simulink model "L3_POLI_ZEROURI_DISCRET"  (R2025b)
settings: Solver=FixedStepDiscrete  StartTime=0.0  StopTime=20  FixedStep=0.1  RelTol=1e-3
settings Model: Creator=elisa  LastModifiedBy=elisa

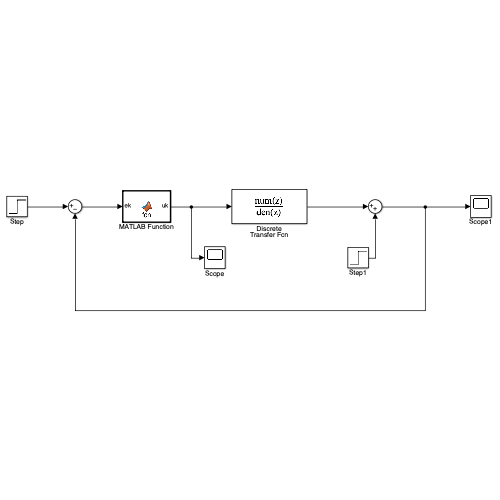
[thumbnail: Simulink's stored preview of the top-level diagram]
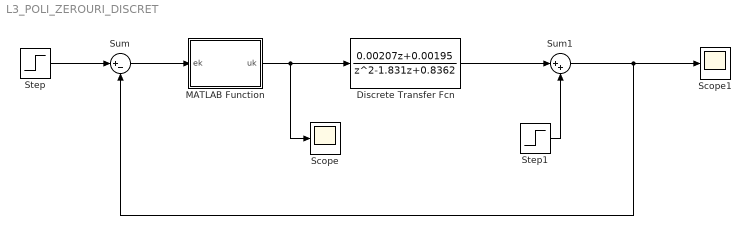
== system L3_POLI_ZEROURI_DISCRET ==
  Discrete Transfer Fcn : DiscreteTransferFcn  Numerator=[0.00207 0.00195]  Denominator=[1 -1.831 0.8362]
  MATLAB Function : MATLAB Function  TreatAsAtomicUnit=on
  Scope : Scope
      settings: ActiveDisplayYMinimum=124.44458746450584  ActiveDisplayYMaximum=170.78058144450188
  Scope1 : Scope
      settings: ActiveDisplayYMinimum=-2.7858479065643103  ActiveDisplayYMaximum=125.07263115907882
  Step : Step  Time=0  After=110  SampleTime=0.1
  Step1 : Step  Time=0  After=10  SampleTime=0.1
  Sum : Sum  Inputs=|+-
  Sum1 : Sum  Inputs=|++
  wires:
  Step/1 -> Sum/1
  Sum/1 -> MATLAB Function/1(ek)
  MATLAB Function/1(uk) -> Scope/1, Discrete Transfer Fcn/1
  Discrete Transfer Fcn/1 -> Sum1/1
  Step1/1 -> Sum1/2
  Sum1/1 -> Sum/2, Scope1/1

== matlab function L3_POLI_ZEROURI_DISCRET/MATLAB Function ==
  data: ek input; uk output

function uk = fcn(ek)

persistent uk_1 ek_1

if isempty(uk_1)
    uk_1 = 0;
    ek_1 = 0;
end

% Regulator PI discret, Kp = 1.3
uk = uk_1 + 1.32964652*ek - 1.27035348*ek_1;

% Actualizarea valorilor
uk_1 = uk;
ek_1 = ek;

end
